simulink model "system"  (R2023a)
settings: Solver=VariableStepAuto  StartTime=0.0  StopTime=15  MaxStep=1E-2  RelTol=1e-3
libraries: fl_lib x6, nesl_utility x3, slpidlib x2, ee_lib x1
settings Model: Creator=delto  LastModifiedBy=LENOVO
settings DataIOCC: SignalLogging=off  DSMLogging=off  ReturnWorkspaceOutputs=off  TimeSaveName=t
settings DebuggingCC: AlgebraicLoopMsg=none  ArtificialAlgebraicLoopMsg=none  ModelReferenceExtraNoncontSigs=none  OperatingPointInterfaceChecksumMismatchMsg=none

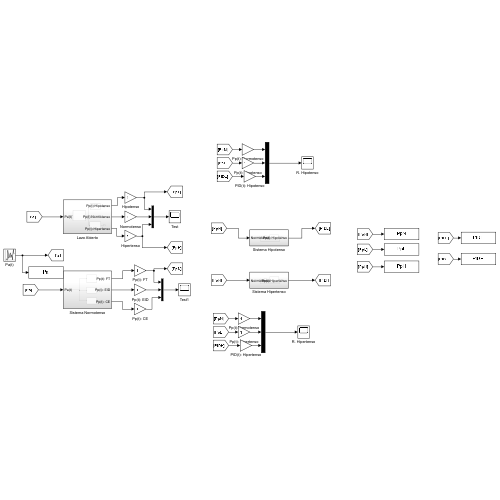
[thumbnail: Simulink's stored preview of the top-level diagram]
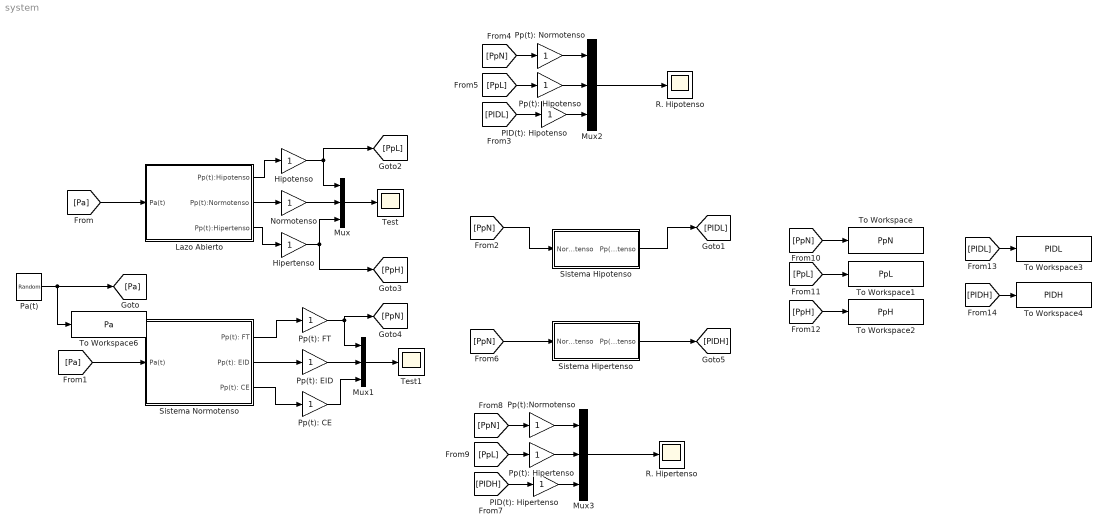
== system system ==
  Hipertenso : Gain
  Hipotenso : Gain
  Lazo Abierto : Subsystem
  Mux{,1..3} (4 alike) : Mux  Inputs=3
  Normotenso : Gain
  PID(t): Hipertenso : Gain
  PID(t): Hipotenso : Gain
  Pa(t) : UniformRandomNumber  SampleTime=0.1
  Pp(t): CE : Gain
  Pp(t): EID : Gain
  Pp(t): FT : Gain
  Pp(t): Hipertenso : Gain
  Pp(t): Hipotenso : Gain
  Pp(t): Normotenso : Gain
  Pp(t):Normotenso : Gain
  R. Hipertenso : Scope
  R. Hipotenso : Scope
  Sistema Hipertenso : Subsystem
  Sistema Hipotenso : Subsystem
  Sistema Normotenso : Subsystem
  Test : Scope
  Test1 : Scope
  To Workspace : ToWorkspace  VariableName=PpN  SampleTime=-1
  To Workspace1 : ToWorkspace  VariableName=PpL  SampleTime=-1
  To Workspace2 : ToWorkspace  VariableName=PpH  SampleTime=-1
  To Workspace3 : ToWorkspace  VariableName=PIDL  SampleTime=-1
  To Workspace4 : ToWorkspace  VariableName=PIDH  SampleTime=-1
  To Workspace6 : ToWorkspace  VariableName=Pa  SampleTime=-1
  wires:
  Pa(t)/1 -> [Pa], To Workspace6/1
  [Pa] -> Lazo Abierto/1(Pa(t))
  Mux/1 -> Test/1
  Hipertenso/1 -> [PpH], Mux/3
  Lazo Abierto/3(Pp(t):Hipertenso) -> Hipertenso/1
  Lazo Abierto/2(Pp(t):Normotenso) -> Normotenso/1
  Lazo Abierto/1(Pp(t):Hipotenso) -> Hipotenso/1
  Hipotenso/1 -> [PpL], Mux/1
  Normotenso/1 -> Mux/2
  [Pa] -> Sistema Normotenso/1(Pa(t))
  Pp(t): FT/1 -> [PpN], Mux1/1
  Mux1/1 -> Test1/1
  Pp(t): CE/1 -> Mux1/3
  Pp(t): EID/1 -> Mux1/2
  Sistema Normotenso/1(Pp(t): FT) -> Pp(t): FT/1
  Sistema Normotenso/2(Pp(t): EID) -> Pp(t): EID/1
  Sistema Normotenso/3(Pp(t): CE) -> Pp(t): CE/1
  [PpN] -> Sistema Hipotenso/1(Normotenso)
  Sistema Hipotenso/1(Pp(t):Hipotenso) -> [PIDL]
  [PpL] -> Pp(t): Hipotenso/1
  [PpN] -> Pp(t): Normotenso/1
  [PIDL] -> PID(t): Hipotenso/1
  Mux2/1 -> R. Hipotenso/1
  Pp(t): Normotenso/1 -> Mux2/1
  Pp(t): Hipotenso/1 -> Mux2/2
  PID(t): Hipotenso/1 -> Mux2/3
  [PpN] -> Sistema Hipertenso/1(Normotenso)
  Sistema Hipertenso/1(Pp(t):Hipertenso) -> [PIDH]
  PID(t): Hipertenso/1 -> Mux3/3
  Pp(t): Hipertenso/1 -> Mux3/2
  Pp(t):Normotenso/1 -> Mux3/1
  Mux3/1 -> R. Hipertenso/1
  [PpN] -> Pp(t):Normotenso/1
  [PpL] -> Pp(t): Hipertenso/1
  [PIDH] -> PID(t): Hipertenso/1
  [PpN] -> To Workspace/1
  [PpL] -> To Workspace1/1
  [PpH] -> To Workspace2/1
  [PIDL] -> To Workspace3/1
  [PIDH] -> To Workspace4/1

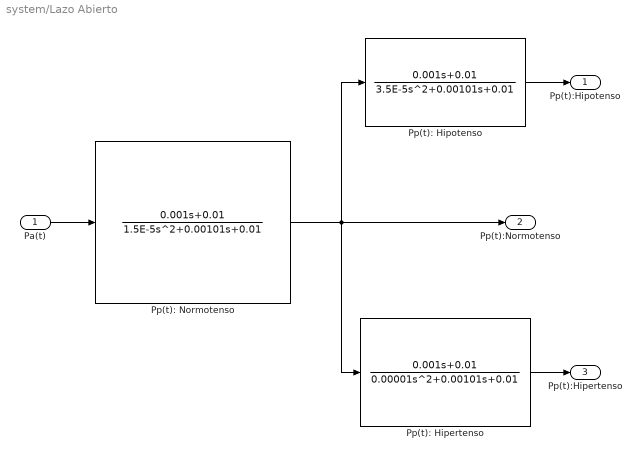
== system system/Lazo Abierto ==
  Pa(t) : Inport
  Pp(t): Hipertenso : TransferFcn  Numerator=[0.001,0.01]  Denominator=[0.00001, 0.00101, 0.01]
  Pp(t): Hipotenso : TransferFcn  Numerator=[0.001,0.01]  Denominator=[3.5E-5, 0.00101, 0.01]
  Pp(t): Normotenso : TransferFcn  Numerator=[0.001,0.01]  Denominator=[1.5E-5, 0.00101, 0.01]
  Pp(t):Hipotenso : Outport
  Pp(t):Normotenso : Outport  Port=2
  Pp(t):Hipertenso : Outport  Port=3
  wires:
  Pa(t)/1 -> Pp(t): Normotenso/1
  Pp(t): Normotenso/1 -> Pp(t): Hipotenso/1, Pp(t): Hipertenso/1, Pp(t):Normotenso/1
  Pp(t): Hipertenso/1 -> Pp(t):Hipertenso/1
  Pp(t): Hipotenso/1 -> Pp(t):Hipotenso/1

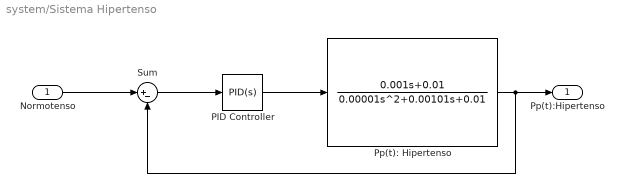
== system system/Sistema Hipertenso ==
  Normotenso : Inport
  PID Controller : slpidlib/PID Controller  Controller=PID  Form=Parallel  TimeDomain=Continuous-time  UseExternalTs=off  SampleTime=-1  IntegratorMethod=Forward Euler  FilterMethod=Forward Euler  ControllerParametersSource=internal  P=1.42831061828755  I=155.70187045244  UseKiTs=off  D=0.00109677996369316  N=259.102823756744  UseFilter=on  TunerSelectOption=Transfer Function Based (PID Tuner App)  InitialConditionSource=internal  InitialConditionForIntegrator=0  InitialConditionForFilter=0  DifferentiatorICPrevScaledInput=0  ExternalReset=none  TrackingMode=off  Kt=1  LimitOutput=off  SatLimitsSource=internal  UpperSaturationLimit=inf  LowerSaturationLimit=-inf  LinearizeAsGain=on  AntiWindupMode=none  Kb=1  LimitIntegrator=off  UpperIntegratorSaturationLimit=inf  LowerIntegratorSaturationLimit=-inf  POutMin=[]  POutMax=[]  IOutMin=[]  IOutMax=[]  DOutMin=[]  DOutMax=[]  NOutMin=[]  NOutMax=[]  SumOutMin=[]  SumOutMax=[]  SaturationOutMin=[]  SaturationOutMax=[]  PParamMin=[]  PParamMax=[]  IParamMin=[]  IParamMax=[]  DParamMin=[]  DParamMax=[]  NParamMin=[]  NParamMax=[]  KbParamMin=[]  KbParamMax=[]  KtParamMin=[]  KtParamMax=[]  KbOutMin=[]  KbOutMax=[]  KtOutMin=[]  KtOutMax=[]  IntegratorOutMin=[]  IntegratorOutMax=[]  FilterOutMin=[]  FilterOutMax=[]  SumI1OutMin=[]  SumI1OutMax=[]  SumI2OutMin=[]  SumI2OutMax=[]  SumI3OutMin=[]  SumI3OutMax=[]  SumI4OutMin=[]  SumI4OutMax=[]  SumDOutMin=[]  SumDOutMax=[]  DifferentiatorOutMin=[]  DifferentiatorOutMax=[]  FilterDiffOutCoefMin=[]  FilterDiffOutCoefMax=[]  ReciprocalOutMin=[]  ReciprocalOutMax=[]  SumDenOutMin=[]  SumDenOutMax=[]  SumNumOutMin=[]  SumNumOutMax=[]  DivideOutMin=[]  DivideOutMax=[]  UdiffTsProdOutMin=[]  UdiffTsProdOutMax=[]  NTsProdOutMin=[]  NTsProdOutMax=[]  UintegralTsProdOutMin=[]  UintegralTsProdOutMax=[]  UngainTsProdOutMin=[]  UngainTsProdOutMax=[]  ClampingZeroOutDataTypeStr=Inherit: Inherit via back propagation  ClampingZeroOutMin=[]  ClampingZeroOutMax=[]  FilterDenConstantOutDataTypeStr=Inherit: Inherit via back propagation  FilterDenConstantOutMin=[]  FilterDenConstantOutMax=[]  PCopyOutDataTypeStr=Inherit: Inherit via back propagation  PCopyOutMin=[]  PCopyOutMax=[]  NCopyOutDataTypeStr=Inherit: Inherit via back propagation  NCopyOutMin=[]  NCopyOutMax=[]  IntegratorContinuousStateAttributes=''  IntegratorStateMustResolveToSignalObject=off  IntegratorRTWStateStorageClass=Auto  FilterContinuousStateAttributes=''  FilterStateMustResolveToSignalObject=off  FilterRTWStateStorageClass=Auto  ParallelPVariant=InternalParameters  IdealPVariant=Disabled  IVariant=InternalParameters  DVariant=InternalParameters  IntegratorVariant=Continuous  SatVariant=Disabled  AWVariant=Passthrough  PCopyVariant=Disabled  TRVariant=Disabled  FdbkBlocksVariant=Forward  IdealPFdbkVariant=Disabled  SatFdbkVariant=Disabled  DerivativeFilterVariant=ContFilter  NVariant=InternalParameters  NCopyVariant=Disabled  FilterICVariant=InternalICsFilter  IntegratorICVariant=InternalICs  ExternalResetVariant=Disabled  TRSumVariant=Passthrough  SumFdbkVariant=Disabled  SumVariant=Sum_PID  TsampFilterVariant=InternalTs  TsampNgainVariant=Passthrough  TsampIntegralVariant=Disabled_SignalSpec  ExternalSaturationOutDataTypeStr=Inherit: Same as second input
  Pp(t): Hipertenso : TransferFcn  Numerator=[0.001,0.01]  Denominator=[0.00001, 0.00101, 0.01]
  Sum : Sum  Inputs=|+-
  Pp(t):Hipertenso : Outport
  wires:
  Normotenso/1 -> Sum/1
  PID Controller/1 -> Pp(t): Hipertenso/1
  Pp(t): Hipertenso/1 -> Sum/2, Pp(t):Hipertenso/1
  Sum/1 -> PID Controller/1

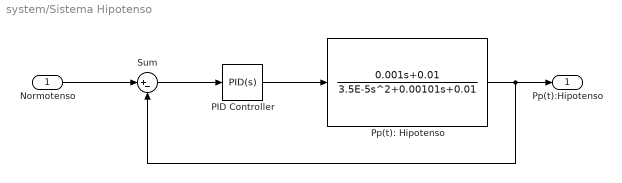
== system system/Sistema Hipotenso ==
  Normotenso : Inport
  PID Controller : slpidlib/PID Controller  Controller=PID  Form=Parallel  TimeDomain=Continuous-time  UseExternalTs=off  SampleTime=-1  IntegratorMethod=Forward Euler  FilterMethod=Forward Euler  ControllerParametersSource=internal  P=291.976430518119  I=451014.46273679  UseKiTs=off  D=0.00626523346028193  N=31877.8327514948  UseFilter=on  TunerSelectOption=Transfer Function Based (PID Tuner App)  InitialConditionSource=internal  InitialConditionForIntegrator=0  InitialConditionForFilter=0  DifferentiatorICPrevScaledInput=0  ExternalReset=none  TrackingMode=off  Kt=1  LimitOutput=off  SatLimitsSource=internal  UpperSaturationLimit=inf  LowerSaturationLimit=-inf  LinearizeAsGain=on  AntiWindupMode=none  Kb=1  LimitIntegrator=off  UpperIntegratorSaturationLimit=inf  LowerIntegratorSaturationLimit=-inf  POutMin=[]  POutMax=[]  IOutMin=[]  IOutMax=[]  DOutMin=[]  DOutMax=[]  NOutMin=[]  NOutMax=[]  SumOutMin=[]  SumOutMax=[]  SaturationOutMin=[]  SaturationOutMax=[]  PParamMin=[]  PParamMax=[]  IParamMin=[]  IParamMax=[]  DParamMin=[]  DParamMax=[]  NParamMin=[]  NParamMax=[]  KbParamMin=[]  KbParamMax=[]  KtParamMin=[]  KtParamMax=[]  KbOutMin=[]  KbOutMax=[]  KtOutMin=[]  KtOutMax=[]  IntegratorOutMin=[]  IntegratorOutMax=[]  FilterOutMin=[]  FilterOutMax=[]  SumI1OutMin=[]  SumI1OutMax=[]  SumI2OutMin=[]  SumI2OutMax=[]  SumI3OutMin=[]  SumI3OutMax=[]  SumI4OutMin=[]  SumI4OutMax=[]  SumDOutMin=[]  SumDOutMax=[]  DifferentiatorOutMin=[]  DifferentiatorOutMax=[]  FilterDiffOutCoefMin=[]  FilterDiffOutCoefMax=[]  ReciprocalOutMin=[]  ReciprocalOutMax=[]  SumDenOutMin=[]  SumDenOutMax=[]  SumNumOutMin=[]  SumNumOutMax=[]  DivideOutMin=[]  DivideOutMax=[]  UdiffTsProdOutMin=[]  UdiffTsProdOutMax=[]  NTsProdOutMin=[]  NTsProdOutMax=[]  UintegralTsProdOutMin=[]  UintegralTsProdOutMax=[]  UngainTsProdOutMin=[]  UngainTsProdOutMax=[]  ClampingZeroOutDataTypeStr=Inherit: Inherit via back propagation  ClampingZeroOutMin=[]  ClampingZeroOutMax=[]  FilterDenConstantOutDataTypeStr=Inherit: Inherit via back propagation  FilterDenConstantOutMin=[]  FilterDenConstantOutMax=[]  PCopyOutDataTypeStr=Inherit: Inherit via back propagation  PCopyOutMin=[]  PCopyOutMax=[]  NCopyOutDataTypeStr=Inherit: Inherit via back propagation  NCopyOutMin=[]  NCopyOutMax=[]  IntegratorContinuousStateAttributes=''  IntegratorStateMustResolveToSignalObject=off  IntegratorRTWStateStorageClass=Auto  FilterContinuousStateAttributes=''  FilterStateMustResolveToSignalObject=off  FilterRTWStateStorageClass=Auto  ParallelPVariant=InternalParameters  IdealPVariant=Disabled  IVariant=InternalParameters  DVariant=InternalParameters  IntegratorVariant=Continuous  SatVariant=Disabled  AWVariant=Passthrough  PCopyVariant=Disabled  TRVariant=Disabled  FdbkBlocksVariant=Forward  IdealPFdbkVariant=Disabled  SatFdbkVariant=Disabled  DerivativeFilterVariant=ContFilter  NVariant=InternalParameters  NCopyVariant=Disabled  FilterICVariant=InternalICsFilter  IntegratorICVariant=InternalICs  ExternalResetVariant=Disabled  TRSumVariant=Passthrough  SumFdbkVariant=Disabled  SumVariant=Sum_PID  TsampFilterVariant=InternalTs  TsampNgainVariant=Passthrough  TsampIntegralVariant=Disabled_SignalSpec  ExternalSaturationOutDataTypeStr=Inherit: Same as second input
  Pp(t): Hipotenso : TransferFcn  Numerator=[0.001,0.01]  Denominator=[3.5E-5, 0.00101, 0.01]
  Sum : Sum  Inputs=|+-
  Pp(t):Hipotenso : Outport
  wires:
  Normotenso/1 -> Sum/1
  PID Controller/1 -> Pp(t): Hipotenso/1
  Pp(t): Hipotenso/1 -> Sum/2, Pp(t):Hipotenso/1
  Sum/1 -> PID Controller/1

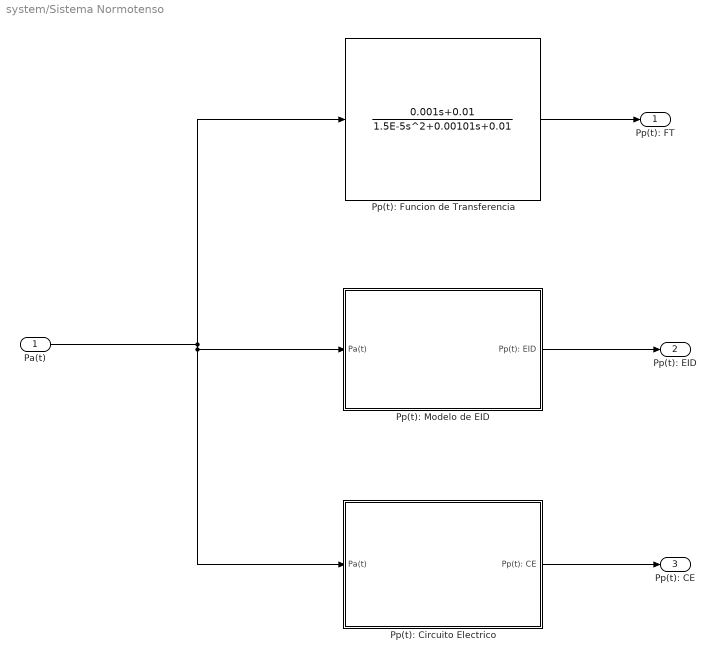
== system system/Sistema Normotenso ==
  Pa(t) : Inport
  Pp(t): Circuito Electrico : Subsystem
  Pp(t): Funcion de Transferencia : TransferFcn  Numerator=[0.001,0.01]  Denominator=[1.5E-5, 0.00101, 0.01]
  Pp(t): Modelo de EID : Subsystem
  Pp(t): FT : Outport
  Pp(t): EID : Outport  Port=2
  Pp(t): CE : Outport  Port=3
  wires:
  Pa(t)/1 -> Pp(t): Modelo de EID/1(Pa(t)), Pp(t): Circuito Electrico/1(Pa(t)), Pp(t): Funcion de Transferencia/1
  Pp(t): Funcion de Transferencia/1 -> Pp(t): FT/1
  Pp(t): Modelo de EID/1(Pp(t): EID) -> Pp(t): EID/1
  Pp(t): Circuito Electrico/1(Pp(t): CE) -> Pp(t): CE/1

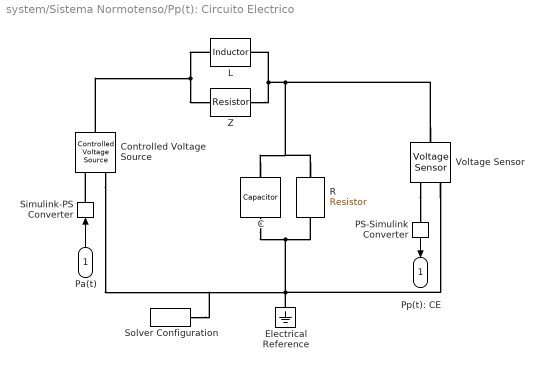
== system system/Sistema Normotenso/Pp(t): Circuito Electrico ==
  Pa(t) : Inport
  C : ee_lib/Passive/Capacitor  cap_option=ee.enum.passive.capacitor.capOption.const  c=1.500 F  Cvec=[1e-05, 1e-06] F  Vvec=[0, 10] V  CV_table_symmetry=ee.enum.passive.capacitor.tableSymmetry.yes  f_vec=[1, 10] kHz  DFext_vec=[.8, 1.2]  enable_C_tol=ee.enum.toleranceApplication.none  averaging_period=0 s  C_tol=5  tol_distribution=ee.enum.toleranceDistribution.uniform  nSigma=4  r=1e-6 Ohm  g=0 1/Ohm  enable_operating_limits=ee.enum.enable.no  enable_faults=ee.enum.enable.no  fault_action=simscape.enum.assert.action.none  Cscale_faulted=100  R_faulted=1e-3 Ohm  G_faulted=0 1/Ohm  tau_fault=1e-3 s  fault_trigger=ee.enum.faults.faultTrigger.temporal  t_fault=1 s  max_permissible_voltage_range=[-100, 100] V  t_fail_on_voltage=1 s  operating_limit_action=ee.enum.passive.reportOpLim.warn  max_working_voltage_range=[-25, 25] V  power_rating=1 W  i_specify=off  i_priority=None  i=0 A  i_nominal_specify=off  i_nominal_unit=A  i_nominal_value=1  v_specify=off  v_priority=None  v=0 V  v_nominal_specify=off  v_nominal_unit=V  v_nominal_value=1  vc_specify=off  vc_priority=High  vc=0 V  vc_nominal_specify=off  vc_nominal_unit=V  vc_nominal_value=1
  Controlled Voltage Source : fl_lib/Electrical/Electrical Sources/Controlled Voltage Source
  Electrical Reference : fl_lib/Electrical/Electrical Elements/Electrical Reference
  L : fl_lib/Electrical/Electrical Elements/Inductor  l=0.001 H  r=0 Ohm  g=1e-9 1/Ohm  i_specify=off  i_priority=None  i=0 A  i_nominal_specify=off  i_nominal_unit=A  i_nominal_value=1  v_specify=off  v_priority=None  v=0 V  v_nominal_specify=off  v_nominal_unit=V  v_nominal_value=1  i_L_specify=off  i_L_priority=High  i_L=0 A  i_L_nominal_specify=off  i_L_nominal_unit=A  i_L_nominal_value=1
  PS-Simulink Converter : nesl_utility/PS-Simulink Converter  PhysicalDomain=network_engine_domain  SubClassName=ps_output  LeftPortType=input  RightPortType=output  PseudoPeriodic=off  Frequencies=[]  VectorFormat=inherit  Unit=inherit  AffineConversion=off
  R : fl_lib/Electrical/Electrical Elements/Resistor  R=1 Ohm  i_specify=off  i_priority=None  i=0 A  i_nominal_specify=off  i_nominal_unit=A  i_nominal_value=1  v_specify=off  v_priority=None  v=0 V  v_nominal_specify=off  v_nominal_unit=V  v_nominal_value=1
  Simulink-PS Converter : nesl_utility/Simulink-PS Converter  PhysicalDomain=network_engine_domain  SubClassName=ps_input  LeftPortType=input  RightPortType=output  PseudoPeriodic=off  Frequencies=[]  NoiseDistribution=none  NoiseParameters=[]  Unit=1  AffineConversion=off  FilteringAndDerivatives=provide  SimscapeFilterOrder=1  InputFilterTimeConstant=0.001  UdotUserProvided=0
  Solver Configuration : nesl_utility/Solver Configuration  PhysicalDomain=network_engine_domain  SubClassName=solver  LeftPortType=input  RightPortType=generic  Tones=[]  Harmonics=[]  SimulateNoise=off  Profile=off  UseLocalSampling=off  EnableSwitchedLinearOptims=on  FrequencyDomain=off  UseCCode=off  RelTol=0.001  AbsTol=0.001  MinStep=1e-09  ToWorkspace=off  RevertToSquareIcSolve=off  NumHomotopyIterations=100  PhasorMode=off  PhasorModeNumHarmonics=1  ConsistencySolver=NEWTON_XTOL_AFTER_FTOL  IndexReductionMethod=DerivativeReplacement  DoDC=off  ResidualTolerance=1e-09  ConsistencyTolSource=GLOBAL  ConsistencyAbsTol=0.001  ConsistencyRelTol=0.001  ConsistencyTolFactor=0.001  UseLocalSolver=off  LocalSolverChoice=NE_BACKWARD_EULER_ADVANCER  ResolveIndetEquations=on  FunctionEvalNumThread=1  LocalSolverSampleTime=0.001  DoFixedCost=off  MaxNonlinIter=3  MaxModeIter=2  ComputeImpulses=off  ImpulseIterations=2  LinearAlgebra=auto  LinearAlgebraNumThread=0  EquationFormulation=NE_TIME_EF  DelaysMemoryBudget=1024  AutomaticFiltering=on  FilteringTimeConstant=0.001  PartitionStorageMethod=AS_NEEDED  PartitionMemoryBudget=1024  PartitionMethod=ROBUST
  Voltage Sensor : fl_lib/Electrical/Electrical Sensors/Voltage Sensor
  Z : fl_lib/Electrical/Electrical Elements/Resistor  R=0.010 Ohm  i_specify=off  i_priority=None  i=0 A  i_nominal_specify=off  i_nominal_unit=A  i_nominal_value=1  v_specify=off  v_priority=None  v=0 V  v_nominal_specify=off  v_nominal_unit=V  v_nominal_value=1
  Pp(t): CE : Outport
  wires:
  Pa(t)/1 -> Simulink-PS Converter/1
  PS-Simulink Converter/1 -> Pp(t): CE/1
  connections:
  L/LConn1 -- Controlled Voltage Source/LConn1 -- Z/LConn1
  C/RConn1 -- Solver Configuration/RConn1 -- Controlled Voltage Source/RConn2 -- Electrical Reference/LConn1 -- Voltage Sensor/RConn2 -- R/RConn1
  Simulink-PS Converter/RConn1 -- Controlled Voltage Source/RConn1
  Voltage Sensor/RConn1 -- PS-Simulink Converter/LConn1
  Voltage Sensor/LConn1 -- C/LConn1 -- R/LConn1 -- Z/RConn1 -- L/RConn1

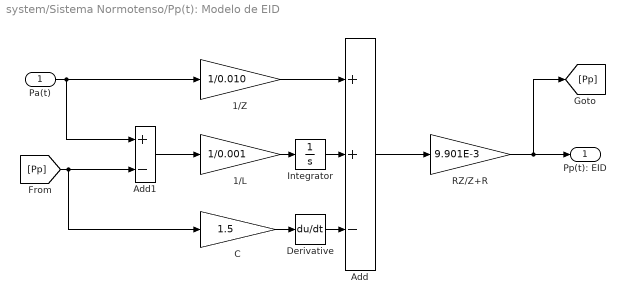
== system system/Sistema Normotenso/Pp(t): Modelo de EID ==
  Pa(t) : Inport
  1/L : Gain  Gain=1/0.001
  1/Z : Gain  Gain=1/0.010
  Add : Sum  Inputs=++-
  Add1 : Sum  Inputs=+-
  C : Gain  Gain=1.5
  Derivative : Derivative
  Integrator : Integrator
  RZ/Z+R : Gain  Gain=9.901E-3
  Pp(t): EID : Outport
  wires:
  Add/1 -> RZ/Z+R/1
  RZ/Z+R/1 -> [Pp], Pp(t): EID/1
  Pa(t)/1 -> Add1/1, 1/Z/1
  1/Z/1 -> Add/1
  [Pp] -> Add1/2, C/1
  Add1/1 -> 1/L/1
  1/L/1 -> Integrator/1
  Integrator/1 -> Add/2
  Derivative/1 -> Add/3
  C/1 -> Derivative/1
